simulink model "kay1024_recursive_demo"  (R2021b)
settings: Solver=FixedStepDiscrete  StartTime=0.0  StopTime=420  FixedStep=1  RelTol=1e-3
InitFcn:
  | kay_demo_init;
undefined symbols (not defined in the file or in its folder): i
libraries: hdlBasic x1189, dspsrcs4 x16, vmcUtilities x1
(part 1 of 14)
settings Model: Creator=Administrator  LastModifiedBy=Administrator

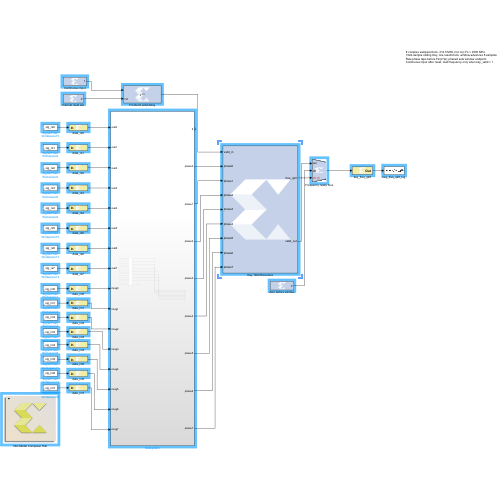
[thumbnail: Simulink's stored preview of the top-level diagram]
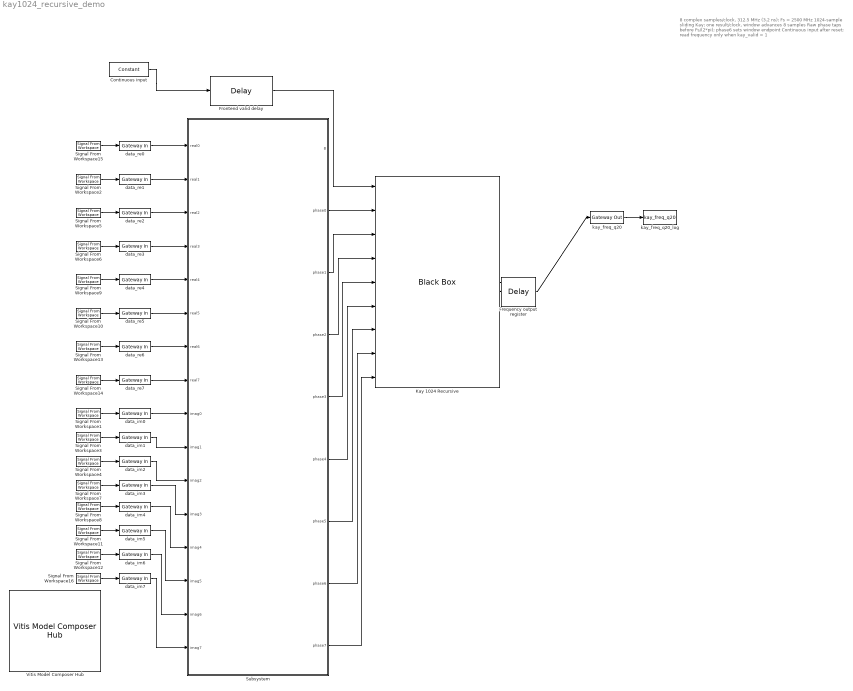
== system kay1024_recursive_demo ==
  note: 8 complex samples/clock, 312.5 MHz (3.2 ns); Fs = 2500 MHz
      | 1024-sample sliding Kay; one result/clock, window advances 8 samples
      | Raw phase taps before Fs/(2*pi); phase6 sets window endpoint
      | Continuous input after reset; read frequency only when kay_valid = 1
  Continuous input : hdlBasic/Constant  const=1  gui_display_data_type=Boolean  arith_type=Boolean  n_bits=16  bin_pt=14  preci_type=Single  exp_width=8  frac_width=24  explicit_period=on  period=1  XmcBlockStatus=1  maskContainerNames=tabcontainer1  block_type=constant  block_config=sysgen:Constant_config
  Frequency output register : hdlBasic/Delay  rst=off  en=off  latency=1  reg_retiming=off  XmcBlockStatus=1  maskContainerNames=group1  block_type=delay  block_config=sysgen:Delay_config
  Frontend valid delay : hdlBasic/Delay  rst=off  en=off  latency=23  reg_retiming=off  XmcBlockStatus=1  maskContainerNames=group1  block_type=delay  block_config=sysgen:Delay_config
  Kay 1024 Recursive : hdlBasic/Black Box  init_code=kay1024_phase_blackbox_config  sim_method=Vivado Simulator  verbose=off  XmcBlockStatus=1  maskContainerNames=group1  block_type=blackbox2  block_config=sysgen:black_box_config
  Signal From Workspace1 : dspsrcs4/Signal From Workspace  X=sig_im0  Ts=1  nsamps=1  OutputAfterFinalValue=Setting to zero  ignoreOrWarnInputAndFrameLengths=off  OutputFrames=on
  Signal From Workspace10 : dspsrcs4/Signal From Workspace  X=sig_re5  Ts=1  nsamps=1  OutputAfterFinalValue=Setting to zero  ignoreOrWarnInputAndFrameLengths=off  OutputFrames=on
  Signal From Workspace11 : dspsrcs4/Signal From Workspace  X=sig_im5  Ts=1  nsamps=1  OutputAfterFinalValue=Setting to zero  ignoreOrWarnInputAndFrameLengths=off  OutputFrames=on
  Signal From Workspace12 : dspsrcs4/Signal From Workspace  X=sig_im6  Ts=1  nsamps=1  OutputAfterFinalValue=Setting to zero  ignoreOrWarnInputAndFrameLengths=off  OutputFrames=on
  Signal From Workspace13 : dspsrcs4/Signal From Workspace  X=sig_re6  Ts=1  nsamps=1  OutputAfterFinalValue=Setting to zero  ignoreOrWarnInputAndFrameLengths=off  OutputFrames=on
  Signal From Workspace14 : dspsrcs4/Signal From Workspace  X=sig_re7  Ts=1  nsamps=1  OutputAfterFinalValue=Setting to zero  ignoreOrWarnInputAndFrameLengths=off  OutputFrames=on
  Signal From Workspace15 : dspsrcs4/Signal From Workspace  X=sig_re0  Ts=1  nsamps=1  OutputAfterFinalValue=Setting to zero  ignoreOrWarnInputAndFrameLengths=off  OutputFrames=on
  Signal From Workspace16 : dspsrcs4/Signal From Workspace  X=sig_im7  Ts=1  nsamps=1  OutputAfterFinalValue=Setting to zero  ignoreOrWarnInputAndFrameLengths=off  OutputFrames=on
  Signal From Workspace2 : dspsrcs4/Signal From Workspace  X=sig_re1  Ts=1  nsamps=1  OutputAfterFinalValue=Setting to zero  ignoreOrWarnInputAndFrameLengths=off  OutputFrames=on
  Signal From Workspace3 : dspsrcs4/Signal From Workspace  X=sig_im1  Ts=1  nsamps=1  OutputAfterFinalValue=Setting to zero  ignoreOrWarnInputAndFrameLengths=off  OutputFrames=on
  Signal From Workspace4 : dspsrcs4/Signal From Workspace  X=sig_im2  Ts=1  nsamps=1  OutputAfterFinalValue=Setting to zero  ignoreOrWarnInputAndFrameLengths=off  OutputFrames=on
  Signal From Workspace5 : dspsrcs4/Signal From Workspace  X=sig_re2  Ts=1  nsamps=1  OutputAfterFinalValue=Setting to zero  ignoreOrWarnInputAndFrameLengths=off  OutputFrames=on
  Signal From Workspace6 : dspsrcs4/Signal From Workspace  X=sig_re3  Ts=1  nsamps=1  OutputAfterFinalValue=Setting to zero  ignoreOrWarnInputAndFrameLengths=off  OutputFrames=on
  Signal From Workspace7 : dspsrcs4/Signal From Workspace  X=sig_im3  Ts=1  nsamps=1  OutputAfterFinalValue=Setting to zero  ignoreOrWarnInputAndFrameLengths=off  OutputFrames=on
  Signal From Workspace8 : dspsrcs4/Signal From Workspace  X=sig_im4  Ts=1  nsamps=1  OutputAfterFinalValue=Setting to zero  ignoreOrWarnInputAndFrameLengths=off  OutputFrames=on
  Signal From Workspace9 : dspsrcs4/Signal From Workspace  X=sig_re4  Ts=1  nsamps=1  OutputAfterFinalValue=Setting to zero  ignoreOrWarnInputAndFrameLengths=off  OutputFrames=on
  Subsystem : Subsystem
  Vitis Model Composer Hub : vmcUtilities/Vitis Model Composer Hub  Tag=genX  CodeGeneration=off  TargetDirectory=E:\FPGA\kay_recursive\build\sysgen  ExportType=System Generator  IpVendor=xilinx.com  IpLibrary=hls  IpVersion=1.0  IpHWLanguage=Verilog  AieCompilerOptions={}  CreateTestbench=off  TestbenchStackSize=10  RunAieSim=off  AieSimTimeout=50000  RunAieSimProfiling=off  LaunchVitisAnalyzer=off  PlotOutput=off  RunX86Sim=off  X86SimTimeout=10  GenHwImage=off  PlatformType=Not Specified  HwSystemType=Baremetal  HwValidationTarget=hw  ProjDevice=xczu47dr-ffve1156-2-i  ProjDevicePart=xczu47dr-ffve1156-2-i  SamplePeriod=-1  ClockFrequency=312.5  DataPathParallelism=1  xilinxfamily=zynquplusRFSOC  part=xczu47dr  speed=-2-i  package=ffve1156  directory=E:\FPGA\kay_recursive\build\sysgen  testbench=off  incr_netlist=off  synthesis_tool=Vivado  clock_wrapper=Clock Enables  dbl_ovrd=According to Block Masks  dcm_input_clock_period=10  sysclk_period=3.2  simulink_period=1  eval_field=0  IPInfoJsonString="{\"HDLSubsystem\":{\"SubsystemName\":\"kay1024_recursive_demo\",\"IPName\":\"kay1024_recursive\",\"IPLibrary\":\"user\",\"IPVendor\":\"user\",\"IPVersion\":\"1.0\"}}"
  data_im{0..7} (8 alike) : hdlBasic/Gateway In  gui_display_data_type=Fixed-point  arith_type=Signed (2's comp)  n_bits=14  bin_pt=13  preci_type=Single  exp_width=8  frac_width=24  rows=1  columns=1  quantization="Round  (unbiased: +/- Inf)"  overflow=Saturate  period=1  UseAsADC=off  ADCChannel='1'  interface=None  automatic_assignment=on  address_offset=hex2dec('00')  intf_name=''  intf_description=''  default_value=0  timing_constraint=None  locs_specified=off  LOCs={}  io_standard={}  inherit_from_input=off  hdl_port=on  XmcBlockStatus=1  maskContainerNames=group4  block_type=gatewayin  block_config=sysgen:gateway_in_config  block_width_w=590  block_height_w=620  block_width=640  block_height=850
  data_re{0..7} (8 alike) : hdlBasic/Gateway In  gui_display_data_type=Fixed-point  arith_type=Signed (2's comp)  n_bits=14  bin_pt=13  preci_type=Single  exp_width=8  frac_width=24  rows=1  columns=1  quantization="Round  (unbiased: +/- Inf)"  overflow=Saturate  period=1  UseAsADC=off  ADCChannel='1'  interface=None  automatic_assignment=on  address_offset=hex2dec('00')  intf_name=''  intf_description=''  default_value=0  timing_constraint=None  locs_specified=off  LOCs={}  io_standard={}  inherit_from_input=off  hdl_port=on  XmcBlockStatus=1  maskContainerNames=group4  block_type=gatewayin  block_config=sysgen:gateway_in_config  block_width_w=590  block_height_w=620  block_width=640  block_height=850
  kay_freq_q20 : hdlBasic/Gateway Out  inherit_from_input=off  hdl_port=on  rows=1  columns=1  UseAsDAC=off  DACChannel='1'  interface=None  automatic_assignment=on  address_offset=hex2dec('00')  intf_name=''  intf_description=''  timing_constraint=None  locs_specified=off  LOCs={}  io_standard={}  XmcBlockStatus=1  maskContainerNames=group4  block_type=gatewayout  block_config=sysgen:gateway_out_config  block_width_w=590  block_height_w=620  block_width=620  block_height=750
  kay_freq_q20_log : ToWorkspace  VariableName=kay_freq_q20  SaveFormat=Timeseries  SampleTime=-1
  wires:
  Subsystem/4(phase2) -> Kay 1024 Recursive/4
  Continuous input/1 -> Frontend valid delay/1
  Frequency output register/1 -> kay_freq_q20/1
  Signal From Workspace6/1 -> data_re3/1
  Subsystem/9(phase7) -> Kay 1024 Recursive/9
  Subsystem/5(phase3) -> Kay 1024 Recursive/5
  data_re1/1 -> Subsystem/2(real1)
  data_im5/1 -> Subsystem/14(imag5)
  Frontend valid delay/1 -> Kay 1024 Recursive/1
  Subsystem/7(phase5) -> Kay 1024 Recursive/7
  Subsystem/3(phase1) -> Kay 1024 Recursive/3
  Signal From Workspace9/1 -> data_re4/1
  Subsystem/8(phase6) -> Kay 1024 Recursive/8
  Signal From Workspace12/1 -> data_im6/1
  Signal From Workspace8/1 -> data_im4/1
  Subsystem/6(phase4) -> Kay 1024 Recursive/6
  Signal From Workspace2/1 -> data_re1/1
  Signal From Workspace13/1 -> data_re6/1
  Signal From Workspace1/1 -> data_im0/1
  Signal From Workspace5/1 -> data_re2/1
  kay_freq_q20/1 -> kay_freq_q20_log/1
  data_re0/1 -> Subsystem/1(real0)
  data_re3/1 -> Subsystem/4(real3)
  Signal From Workspace7/1 -> data_im3/1
  data_re5/1 -> Subsystem/6(real5)
  data_re6/1 -> Subsystem/7(real6)
  data_im2/1 -> Subsystem/11(imag2)
  data_im7/1 -> Subsystem/16(imag7)
  data_im6/1 -> Subsystem/15(imag6)
  Subsystem/2(phase0) -> Kay 1024 Recursive/2
  data_im3/1 -> Subsystem/12(imag3)
  Signal From Workspace10/1 -> data_re5/1
  Kay 1024 Recursive/1 -> Frequency output register/1
  data_im1/1 -> Subsystem/10(imag1)
  Signal From Workspace16/1 -> data_im7/1
  Signal From Workspace4/1 -> data_im2/1
  data_re4/1 -> Subsystem/5(real4)
  Signal From Workspace3/1 -> data_im1/1
  Signal From Workspace15/1 -> data_re0/1
  Signal From Workspace14/1 -> data_re7/1
  data_re7/1 -> Subsystem/8(real7)
  Signal From Workspace11/1 -> data_im5/1
  data_im0/1 -> Subsystem/9(imag0)
  data_re2/1 -> Subsystem/3(real2)
  data_im4/1 -> Subsystem/13(imag4)

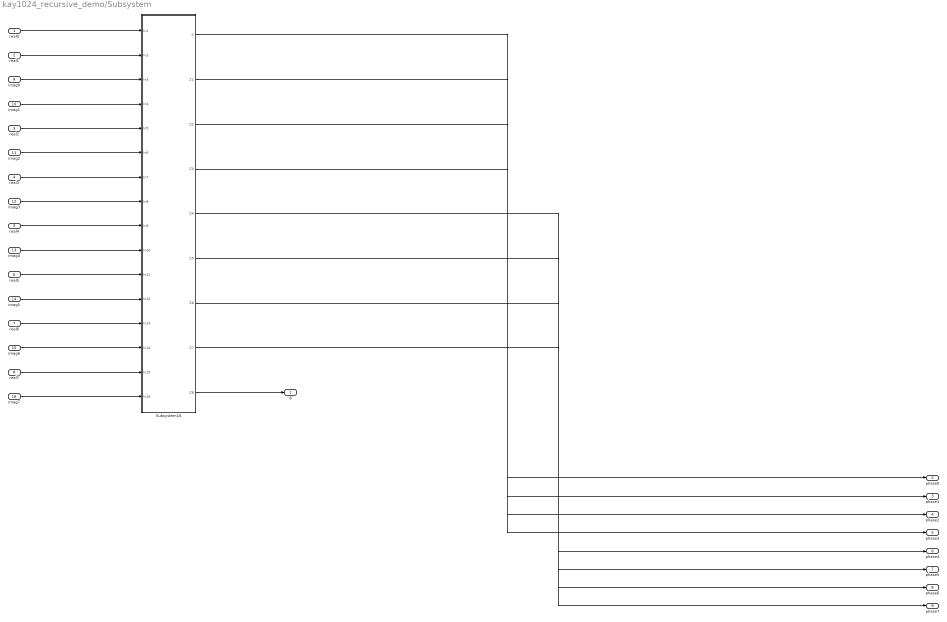
== system kay1024_recursive_demo/Subsystem ==
  real0 : Inport
  real1 : Inport  Port=2
  real2 : Inport  Port=3
  real3 : Inport  Port=4
  real4 : Inport  Port=5
  real5 : Inport  Port=6
  real6 : Inport  Port=7
  real7 : Inport  Port=8
  imag0 : Inport  Port=9
  imag1 : Inport  Port=10
  imag2 : Inport  Port=11
  imag3 : Inport  Port=12
  imag4 : Inport  Port=13
  imag5 : Inport  Port=14
  imag6 : Inport  Port=15
  imag7 : Inport  Port=16
  Subsystem16 : Subsystem
  8 : Outport
  phase0 : Outport  Port=2
  phase1 : Outport  Port=3
  phase2 : Outport  Port=4
  phase3 : Outport  Port=5
  phase4 : Outport  Port=6
  phase5 : Outport  Port=7
  phase6 : Outport  Port=8
  phase7 : Outport  Port=9
  wires:
  real0/1 -> Subsystem16/1(In1)
  real1/1 -> Subsystem16/2(In2)
  imag0/1 -> Subsystem16/3(In3)
  imag1/1 -> Subsystem16/4(In4)
  real2/1 -> Subsystem16/5(In5)
  imag2/1 -> Subsystem16/6(In6)
  real3/1 -> Subsystem16/7(In7)
  imag3/1 -> Subsystem16/8(In8)
  real4/1 -> Subsystem16/9(In9)
  imag4/1 -> Subsystem16/10(In10)
  real5/1 -> Subsystem16/11(In11)
  imag5/1 -> Subsystem16/12(In12)
  real6/1 -> Subsystem16/13(In13)
  imag6/1 -> Subsystem16/14(In14)
  real7/1 -> Subsystem16/15(In15)
  imag7/1 -> Subsystem16/16(In16)
  Subsystem16/8(Z7) -> phase7/1
  Subsystem16/7(Z6) -> phase6/1
  Subsystem16/6(Z5) -> phase5/1
  Subsystem16/5(Z4) -> phase4/1
  Subsystem16/3(Z2) -> phase2/1
  Subsystem16/2(Z1) -> phase1/1
  Subsystem16/4(Z3) -> phase3/1
  Subsystem16/1(Z) -> phase0/1
  Subsystem16/9(Z8) -> 8/1

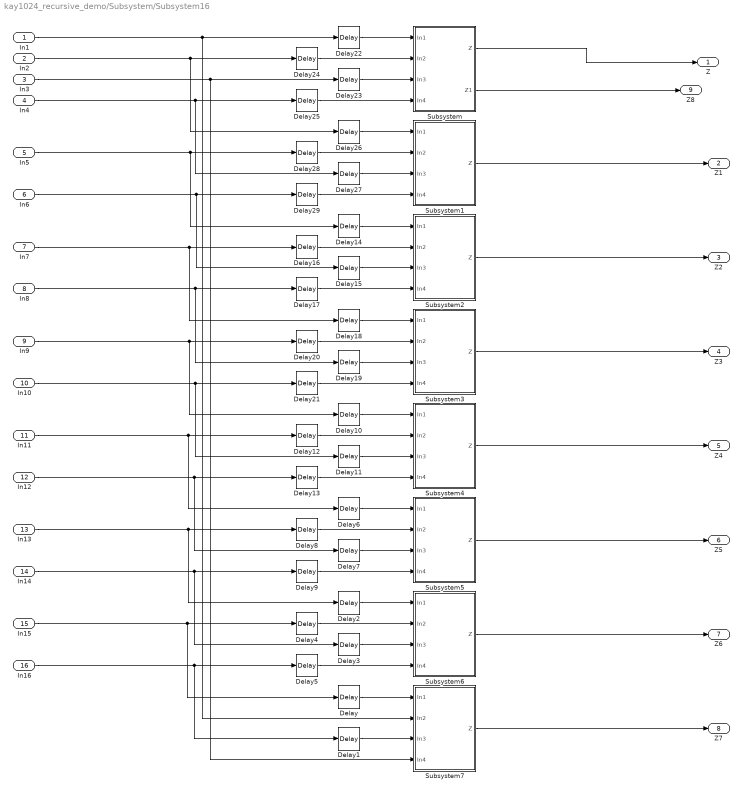
== system kay1024_recursive_demo/Subsystem/Subsystem16 ==
  In1 : Inport
  In2 : Inport  Port=2
  In3 : Inport  Port=3
  In4 : Inport  Port=4
  In5 : Inport  Port=5
  In6 : Inport  Port=6
  In7 : Inport  Port=7
  In8 : Inport  Port=8
  In9 : Inport  Port=9
  In10 : Inport  Port=10
  In11 : Inport  Port=11
  In12 : Inport  Port=12
  In13 : Inport  Port=13
  In14 : Inport  Port=14
  In15 : Inport  Port=15
  In16 : Inport  Port=16
  Delay{,1..29} (30 alike) : hdlBasic/Delay  rst=off  en=off  latency=1  reg_retiming=off  XmcBlockStatus=1  maskContainerNames=group1  block_type=delay  block_config=sysgen:Delay_config
  Subsystem : Subsystem
  Subsystem1 : Subsystem
  Subsystem2 : Subsystem
  Subsystem3 : Subsystem
  Subsystem4 : Subsystem
  Subsystem5 : Subsystem
  Subsystem6 : Subsystem
  Subsystem7 : Subsystem
  Z : Outport
  Z1 : Outport  Port=2
  Z2 : Outport  Port=3
  Z3 : Outport  Port=4
  Z4 : Outport  Port=5
  Z5 : Outport  Port=6
  Z6 : Outport  Port=7
  Z7 : Outport  Port=8
  Z8 : Outport  Port=9
  wires:
  In3/1 -> Subsystem7/4(In4), Delay23/1
  In16/1 -> Delay5/1, Delay1/1
  In1/1 -> Subsystem7/2(In2), Delay22/1
  In11/1 -> Delay12/1, Delay6/1
  In6/1 -> Delay15/1, Delay29/1
  In4/1 -> Delay27/1, Delay25/1
  In13/1 -> Delay2/1, Delay8/1
  In9/1 -> Delay10/1, Delay20/1
  In7/1 -> Delay18/1, Delay16/1
  In8/1 -> Delay19/1, Delay17/1
  In12/1 -> Delay7/1, Delay13/1
  In2/1 -> Delay26/1, Delay24/1
  Subsystem5/1(Z) -> Z5/1
  Subsystem7/1(Z) -> Z7/1
  In5/1 -> Delay14/1, Delay28/1
  Subsystem1/1(Z) -> Z1/1
  In14/1 -> Delay3/1, Delay9/1
  In10/1 -> Delay11/1, Delay21/1
  In15/1 -> Delay4/1, Delay/1
  Subsystem/1(Z) -> Z/1
  Subsystem4/1(Z) -> Z4/1
  Subsystem6/1(Z) -> Z6/1
  Subsystem2/1(Z) -> Z2/1
  Subsystem3/1(Z) -> Z3/1
  Delay/1 -> Subsystem7/1(In1)
  Delay1/1 -> Subsystem7/3(In3)
  Delay3/1 -> Subsystem6/3(In3)
  Delay2/1 -> Subsystem6/1(In1)
  Delay4/1 -> Subsystem6/2(In2)
  Delay5/1 -> Subsystem6/4(In4)
  Delay9/1 -> Subsystem5/4(In4)
  Delay7/1 -> Subsystem5/3(In3)
  Delay8/1 -> Subsystem5/2(In2)
  Delay6/1 -> Subsystem5/1(In1)
  Delay13/1 -> Subsystem4/4(In4)
  Delay10/1 -> Subsystem4/1(In1)
  Delay12/1 -> Subsystem4/2(In2)
  Delay11/1 -> Subsystem4/3(In3)
  Delay15/1 -> Subsystem2/3(In3)
  Delay16/1 -> Subsystem2/2(In2)
  Delay14/1 -> Subsystem2/1(In1)
  Delay21/1 -> Subsystem3/4(In4)
  Delay19/1 -> Subsystem3/3(In3)
  Delay20/1 -> Subsystem3/2(In2)
  Delay17/1 -> Subsystem2/4(In4)
  Delay18/1 -> Subsystem3/1(In1)
  Delay26/1 -> Subsystem1/1(In1)
  Delay27/1 -> Subsystem1/3(In3)
  Delay28/1 -> Subsystem1/2(In2)
  Delay29/1 -> Subsystem1/4(In4)
  Delay23/1 -> Subsystem/3(In3)
  Delay24/1 -> Subsystem/2(In2)
  Delay22/1 -> Subsystem/1(In1)
  Delay25/1 -> Subsystem/4(In4)
  Subsystem/2(Z1) -> Z8/1

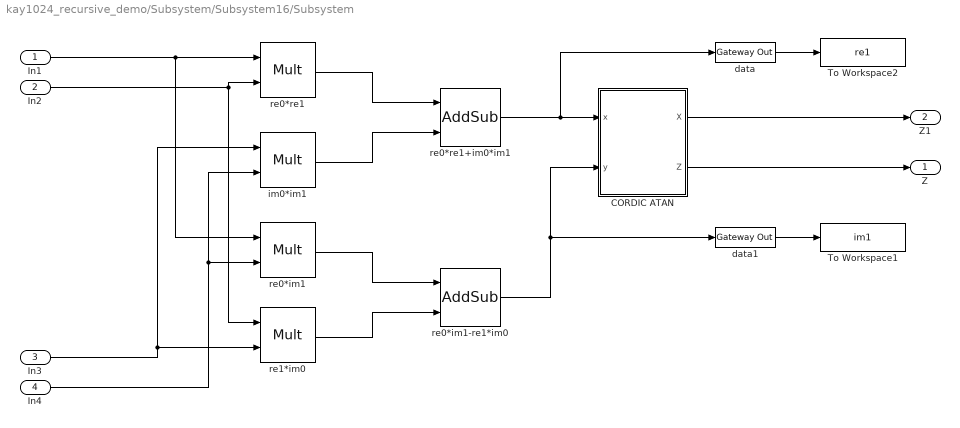
== system kay1024_recursive_demo/Subsystem/Subsystem16/Subsystem ==
  In1 : Inport
  In2 : Inport  Port=2
  In3 : Inport  Port=3
  In4 : Inport  Port=4
  CORDIC ATAN : Subsystem  mask(Xilinx CORDIC ATAN){stages=15, pe_nbits=30, pe_binpt=18, pipeline_x=ones(1,15), prev_stages=15, pipeline=[1  1  1  1  1  1  1  1  1  1  1  1  1  1  1]}
      mask prompts: stages "Number of Processing Elements (integer value starting from 1)"; pe_nbits "X, Y Data Width"; pe_binpt "X, Y Binary Point Position"; pipeline_x "Latency for each Processing Element [1 0 0 1]"; prev_stages "Previous Number of Stages"; pipeline "Previous Pipeline Values"
      mask help: A parallel implementation, circular vectoring mode CORDIC processor for performing rectangular-to-polar conversion. The number of iteration stages (and resultant output accuracy) and the processor arithmetic precision are controlled by the mask customization.
      mask init:
      | [bg,fg] = xlcmap('XBlock',0);
      | iPos = get_param(gcb,'Position');
      | iWidth=iPos(3)-iPos(1); iHeight=iPos(4)-iPos(2);
      | iCx=iWidth/2;
      | iCy=iHeight/2;
      | [logoX, logoY] = xlogo(iPos);
      | sav_gcb=gcb;
      | stages = round(sum(abs(stages)));
      | if (stages == 0)
      | 	stages = prev_stages;
      | end
      | x = zeros(1,stages);
      | pipe_size = max(size(pipeline_x));
      | if pipe_size >= stages
      | 	x(1,1:stages) = pipeline_x(1,1:stages);
      | else
      | 	x(1,1:pipe_size) = pipeline_x(1,1:pipe_size);
      | end
      | 
      | if (stages ~=prev_stages)
      | 	pipeline=x;
      | 	cordic_pe = find_system(gcb, 'lookUnderMasks', 'all', 'FollowLinks','on','masktype', 'CORDIC parallel PE');
      |     
      |   a=find_system(cordic_pe{1}, 'lookUnderMasks', 'all', 'FollowLinks','on','masktype', 'CORDIC iteration PE');
      |   for i= 2:length(a)
      |     for j=1:3
      | 	  delete_line(cordic_pe{1}, ['CORDIC PE' int2str(i-1) '/' int2str(j)], ['CORDIC PE' int2str(i) '/' int2str(j)]);
      |     end
      |   end
      |     if length(a)>0,
      |       delete_line(cordic_pe{1}, 'x/1', 'CORDIC PE1/1');
      |       delete_line(cordic_pe{1}, 'y/1', 'CORDIC PE1/2');
      |       delete_line(cordic_pe{1}, 'z/1', 'CORDIC PE1/3');
      |       delete_line(cordic_pe{1}, ['CORDIC PE' int2str(length(a)) '/1'],'X/1');
      |       delete_line(cordic_pe{1}, ['CORDIC PE' int2str(length(a)) '/2'],'Terminator/1');
      |       delete_line(cordic_pe{1}, ['CORDIC PE' int2str(length(a)) '/3'],'Z/1');
      |     elseif length(a)==0
      |       temp_port=get_param([cordic_pe{1} '/x'],'porthandles');
      |       temp_line=get_param(temp_port.Outport,'line');
      |       if temp_line>=0  delete_line(temp_line); end
      |       temp_port=get_param([cordic_pe{1} '/y'],'porthandles');
      |       temp_line=get_param(temp_port.Outport,'line');
      |       if temp_line>=0  delete_line(temp_line); end
      |       temp_port=get_param([cordic_pe{1} '/z'],'porthandles');
      |       temp_line=get_param(temp_port.Outport,'line');
      |       if temp_line>=0  delete_line(temp_line); end
      |     end
      | 
      |     for i=2:length(a)
      |       delete_block(a{i});
      |     end
      |     for i=2:stages,
      |         add_block([cordic_pe{1} '/CORDIC PE1'], [cordic_pe{1} '/CORDIC PE' int2str(i)], 'ii', int2str(i-1),'pe_nbits', 'pe_nbits','pe_binpt', 'pe_binpt','pipeline',['pipeline(1,' int2str(i) ')'],'position',[150+(i-1)*125, 70, 205+(i-1)*125, 130]);
      |     end
      | 
      |     for i= 2:stages,
      |       for j=1:3
      | 		add_line(cordic_pe{1}, ['CORDIC PE' int2str(i-1) '/' int2str(j)], ['CORDIC PE' int2str(i) '/' int2str(j)], 'autorouting', 'on');
      |       end
      |     end
      | 
      |     if stages==0
      |       add_line(cordic_pe{1}, 'x/1', 'X/1', 'autorouting', 'on');
      |       add_line(cordic_pe{1}, 'y/1', 'Terminator/1', 'autorouting', 'on');
      |       add_line(cordic_pe{1}, 'z/1', 'Z/1', 'autorouting', 'on');
      |     elseif stages>0
      |       add_line(cordic_pe{1}, 'x/1', 'CORDIC PE1/1', 'autorouting', 'on');
      |       add_line(cordic_pe{1}, 'y/1', 'CORDIC PE1/2', 'autorouting', 'on');
      |       add_line(cordic_pe{1}, 'z/1', 'CORDIC PE1/3', 'autorouting', 'on');
      | 
      |       set_param([cordic_pe{1} '/' 'X'], 'Position', [150+stages*125, 72, 180+stages*125, 86]);
      |       set_param([cordic_pe{1} '/' 'Terminator'], 'Position', [210+stages*125, 92, 225+stages*125, 108]);
      |       set_param([cordic_pe{1} '/' 'Z'], 'Position', [240+stages*125, 113, 270+stages*125, 127]);
      | 
      |       add_line(cordic_pe{1}, ['CORDIC PE' int2str(stages) '/1'], 'X/1', 'autorouting', 'on');
      |       add_line(cordic_pe{1}, ['CORDIC PE' int2str(stages) '/2'], 'Terminator/1', 'autorouting', 'on');
      |       add_line(cordic_pe{1}, ['CORDIC PE' int2str(stages) '/3'],'Z/1', 'autorouting', 'on');
      | 
      |       % force a "compile" of the constituent constant blocks to
      |       % workaround a data propagation problem
      |       find_system(cordic_pe{1}, 'lookUnderMasks', 'all', 'FollowLinks', 'on', 'MaskType','Xilinx Constant Block');
      |   end
      | 	set_param(sav_gcb, 'prev_stages', int2str(stages));
      | 	set_param(sav_gcb, 'pipeline', [ '[' int2str(x) ']']);
      | else
      | 	if (sum(pipeline~=x))
      | 		set_param(gcb, 'pipeline', [ '[' int2str(x) ']']);
      | 	end
      | end
      | str = sprintf('-%d',sum(x) + 3);
      settings: CopyFcn=set_param(gcb, 'MaskSelfModifiable', 'on', 'LinkStatus', 'none');
      mask Help: eval('');xlDoc('-book','sysgen','-topic','CORDIC_ATAN');
      mask Display:
      | patch([0 iWidth iWidth 0],[0 0 iHeight iHeight] , bg);
      | patch(logoX,logoY , fg);
      | text(iCx-6,iCy,'z');
      | text(iCx,iCy+4,str);
      | port_label('input',1,'x');
      | port_label('input',2,'y');
      | port_label('output',1,'mag');
      | port_label('output',2,'atan');
      | plot([0 0 iWidth iWidth 0], [0 iHeight iHeight 0 0]);
  To Workspace1 : ToWorkspace  VariableName=im1  SampleTime=-1
      settings: Save2DSignal=2-D array (concatenate along first dimension)
  To Workspace2 : ToWorkspace  VariableName=re1  SampleTime=-1
      settings: Save2DSignal=2-D array (concatenate along first dimension)
  data : hdlBasic/Gateway Out  inherit_from_input=on  hdl_port=off  rows=1  columns=1  UseAsDAC=off  DACChannel='1'  interface=None  automatic_assignment=on  address_offset=hex2dec('00')  intf_name=''  intf_description=''  timing_constraint=None  locs_specified=off  LOCs={}  io_standard={}  XmcBlockStatus=1  maskContainerNames=group4  block_type=gatewayout  block_config=sysgen:gateway_out_config  block_width_w=590  block_height_w=620  block_width=620  block_height=750
  data1 : hdlBasic/Gateway Out  inherit_from_input=on  hdl_port=off  rows=1  columns=1  UseAsDAC=off  DACChannel='1'  interface=None  automatic_assignment=on  address_offset=hex2dec('00')  intf_name=''  intf_description=''  timing_constraint=None  locs_specified=off  LOCs={}  io_standard={}  XmcBlockStatus=1  maskContainerNames=group4  block_type=gatewayout  block_config=sysgen:gateway_out_config  block_width_w=590  block_height_w=620  block_width=620  block_height=750
  im0*im1 : hdlBasic/Mult  precision=Full  arith_type="Signed  (2's comp)"  n_bits=16  bin_pt=14  quantization=Truncate  overflow=Wrap  en=off  latency=3  use_behavioral_HDL=off  opt=Speed  use_embedded=on  optimum_pipeline=off  pipeline=on  use_rpm=on  placement_style=Triangular  XmcBlockStatus=1  maskContainerNames=group1  block_type=mult  block_config=sysgen:Mult_config  block_width=598  block_height=876
  re0*im1 : hdlBasic/Mult  precision=Full  arith_type="Signed  (2's comp)"  n_bits=16  bin_pt=14  quantization=Truncate  overflow=Wrap  en=off  latency=3  use_behavioral_HDL=off  opt=Speed  use_embedded=on  optimum_pipeline=off  pipeline=on  use_rpm=on  placement_style=Triangular  XmcBlockStatus=1  maskContainerNames=group1  block_type=mult  block_config=sysgen:Mult_config  block_width=598  block_height=876
  re0*im1-re1*im0 : hdlBasic/AddSub  mode=Subtraction  use_carryin=off  use_carryout=off  en=off  latency=1  precision=Full  arith_type=Unsigned  n_bits=16  bin_pt=14  quantization=Truncate  overflow=Wrap  use_behavioral_HDL=off  hw_selection=Fabric  pipelined=off  XmcBlockStatus=1  maskContainerNames=tabcontainer1  block_type=addsub  block_config=sysgen:Addsub_config
  re0*re1 : hdlBasic/Mult  precision=Full  arith_type="Signed  (2's comp)"  n_bits=16  bin_pt=14  quantization=Truncate  overflow=Wrap  en=off  latency=3  use_behavioral_HDL=off  opt=Speed  use_embedded=on  optimum_pipeline=off  pipeline=on  use_rpm=on  placement_style=Triangular  XmcBlockStatus=1  maskContainerNames=group1  block_type=mult  block_config=sysgen:Mult_config  block_width=598  block_height=876
  re0*re1+im0*im1 : hdlBasic/AddSub  mode=Addition  use_carryin=off  use_carryout=off  en=off  latency=1  precision=Full  arith_type=Unsigned  n_bits=16  bin_pt=14  quantization=Truncate  overflow=Wrap  use_behavioral_HDL=off  hw_selection=Fabric  pipelined=off  XmcBlockStatus=1  maskContainerNames=tabcontainer1  block_type=addsub  block_config=sysgen:Addsub_config
  re1*im0 : hdlBasic/Mult  precision=Full  arith_type="Signed  (2's comp)"  n_bits=16  bin_pt=14  quantization=Truncate  overflow=Wrap  en=off  latency=3  use_behavioral_HDL=off  opt=Speed  use_embedded=on  optimum_pipeline=off  pipeline=on  use_rpm=on  placement_style=Triangular  XmcBlockStatus=1  maskContainerNames=group1  block_type=mult  block_config=sysgen:Mult_config  block_width=598  block_height=876
  Z : Outport
  Z1 : Outport  Port=2
  wires:
  In3/1 -> re1*im0/2, im0*im1/1
  re0*im1-re1*im0/1 -> CORDIC ATAN/2(y), data1/1
  In2/1 -> re0*re1/2, re1*im0/1
  In4/1 -> re0*im1/2, im0*im1/2
  re0*im1/1 -> re0*im1-re1*im0/1
  In1/1 -> re0*im1/1, re0*re1/1
  re0*re1/1 -> re0*re1+im0*im1/1
  im0*im1/1 -> re0*re1+im0*im1/2
  re0*re1+im0*im1/1 -> data/1, CORDIC ATAN/1(x)
  re1*im0/1 -> re0*im1-re1*im0/2
  CORDIC ATAN/2(Z) -> Z/1
  data/1 -> To Workspace2/1
  data1/1 -> To Workspace1/1
  CORDIC ATAN/1(X) -> Z1/1

== system kay1024_recursive_demo/Subsystem/Subsystem16/Subsystem1 ==
  In1 : Inport
  In2 : Inport  Port=2
  In3 : Inport  Port=3
  In4 : Inport  Port=4
  CORDIC ATAN : Subsystem  mask(Xilinx CORDIC ATAN){stages=15, pe_nbits=30, pe_binpt=18, pipeline_x=ones(1,15), prev_stages=15, pipeline=[1  1  1  1  1  1  1  1  1  1  1  1  1  1  1]}
      mask prompts: stages "Number of Processing Elements (integer value starting from 1)"; pe_nbits "X, Y Data Width"; pe_binpt "X, Y Binary Point Position"; pipeline_x "Latency for each Processing Element [1 0 0 1]"; prev_stages "Previous Number of Stages"; pipeline "Previous Pipeline Values"
      mask help: A parallel implementation, circular vectoring mode CORDIC processor for performing rectangular-to-polar conversion. The number of iteration stages (and resultant output accuracy) and the processor arithmetic precision are controlled by the mask customization.
      mask init: same as kay1024_recursive_demo/Subsystem/Subsystem16/Subsystem/CORDIC ATAN
      settings: CopyFcn=set_param(gcb, 'MaskSelfModifiable', 'on', 'LinkStatus', 'none');
      mask Help: eval('');xlDoc('-book','sysgen','-topic','CORDIC_ATAN');
      mask Display:
      | patch([0 iWidth iWidth 0],[0 0 iHeight iHeight] , bg);
      | patch(logoX,logoY , fg);
      | text(iCx-6,iCy,'z');
      | text(iCx,iCy+4,str);
      | port_label('input',1,'x');
      | port_label('input',2,'y');
      | port_label('output',1,'mag');
      | port_label('output',2,'atan');
      | plot([0 0 iWidth iWidth 0], [0 iHeight iHeight 0 0]);
  im0*im1 : hdlBasic/Mult  precision=Full  arith_type="Signed  (2's comp)"  n_bits=16  bin_pt=14  quantization=Truncate  overflow=Wrap  en=off  latency=3  use_behavioral_HDL=off  opt=Speed  use_embedded=on  optimum_pipeline=off  pipeline=on  use_rpm=on  placement_style=Triangular  XmcBlockStatus=1  maskContainerNames=group1  block_type=mult  block_config=sysgen:Mult_config  block_width=598  block_height=876
  re0*im1 : hdlBasic/Mult  precision=Full  arith_type="Signed  (2's comp)"  n_bits=16  bin_pt=14  quantization=Truncate  overflow=Wrap  en=off  latency=3  use_behavioral_HDL=off  opt=Speed  use_embedded=on  optimum_pipeline=off  pipeline=on  use_rpm=on  placement_style=Triangular  XmcBlockStatus=1  maskContainerNames=group1  block_type=mult  block_config=sysgen:Mult_config  block_width=598  block_height=876
  re0*im1-re1*im0 : hdlBasic/AddSub  mode=Subtraction  use_carryin=off  use_carryout=off  en=off  latency=1  precision=Full  arith_type=Unsigned  n_bits=16  bin_pt=14  quantization=Truncate  overflow=Wrap  use_behavioral_HDL=off  hw_selection=Fabric  pipelined=off  XmcBlockStatus=1  maskContainerNames=tabcontainer1  block_type=addsub  block_config=sysgen:Addsub_config
  re0*re1 : hdlBasic/Mult  precision=Full  arith_type="Signed  (2's comp)"  n_bits=16  bin_pt=14  quantization=Truncate  overflow=Wrap  en=off  latency=3  use_behavioral_HDL=off  opt=Speed  use_embedded=on  optimum_pipeline=off  pipeline=on  use_rpm=on  placement_style=Triangular  XmcBlockStatus=1  maskContainerNames=group1  block_type=mult  block_config=sysgen:Mult_config  block_width=598  block_height=876
  re0*re1+im0*im1 : hdlBasic/AddSub  mode=Addition  use_carryin=off  use_carryout=off  en=off  latency=1  precision=Full  arith_type=Unsigned  n_bits=16  bin_pt=14  quantization=Truncate  overflow=Wrap  use_behavioral_HDL=off  hw_selection=Fabric  pipelined=off  XmcBlockStatus=1  maskContainerNames=tabcontainer1  block_type=addsub  block_config=sysgen:Addsub_config
  re1*im0 : hdlBasic/Mult  precision=Full  arith_type="Signed  (2's comp)"  n_bits=16  bin_pt=14  quantization=Truncate  overflow=Wrap  en=off  latency=3  use_behavioral_HDL=off  opt=Speed  use_embedded=on  optimum_pipeline=off  pipeline=on  use_rpm=on  placement_style=Triangular  XmcBlockStatus=1  maskContainerNames=group1  block_type=mult  block_config=sysgen:Mult_config  block_width=598  block_height=876
  Z : Outport
  wires:
  In3/1 -> re1*im0/2, im0*im1/1
  re0*im1-re1*im0/1 -> CORDIC ATAN/2(y)
  In2/1 -> re0*re1/2, re1*im0/1
  In4/1 -> re0*im1/2, im0*im1/2
  re0*im1/1 -> re0*im1-re1*im0/1
  In1/1 -> re0*im1/1, re0*re1/1
  re0*re1/1 -> re0*re1+im0*im1/1
  im0*im1/1 -> re0*re1+im0*im1/2
  re0*re1+im0*im1/1 -> CORDIC ATAN/1(x)
  re1*im0/1 -> re0*im1-re1*im0/2
  CORDIC ATAN/2(Z) -> Z/1

== system kay1024_recursive_demo/Subsystem/Subsystem16/Subsystem2 ==
  In1 : Inport
  In2 : Inport  Port=2
  In3 : Inport  Port=3
  In4 : Inport  Port=4
  CORDIC ATAN : Subsystem  mask(Xilinx CORDIC ATAN){stages=15, pe_nbits=30, pe_binpt=18, pipeline_x=ones(1,15), prev_stages=15, pipeline=[1  1  1  1  1  1  1  1  1  1  1  1  1  1  1]}
      mask prompts: stages "Number of Processing Elements (integer value starting from 1)"; pe_nbits "X, Y Data Width"; pe_binpt "X, Y Binary Point Position"; pipeline_x "Latency for each Processing Element [1 0 0 1]"; prev_stages "Previous Number of Stages"; pipeline "Previous Pipeline Values"
      mask help: A parallel implementation, circular vectoring mode CORDIC processor for performing rectangular-to-polar conversion. The number of iteration stages (and resultant output accuracy) and the processor arithmetic precision are controlled by the mask customization.
      mask init: same as kay1024_recursive_demo/Subsystem/Subsystem16/Subsystem/CORDIC ATAN
      settings: CopyFcn=set_param(gcb, 'MaskSelfModifiable', 'on', 'LinkStatus', 'none');
      mask Help: eval('');xlDoc('-book','sysgen','-topic','CORDIC_ATAN');
      mask Display:
      | patch([0 iWidth iWidth 0],[0 0 iHeight iHeight] , bg);
      | patch(logoX,logoY , fg);
      | text(iCx-6,iCy,'z');
      | text(iCx,iCy+4,str);
      | port_label('input',1,'x');
      | port_label('input',2,'y');
      | port_label('output',1,'mag');
      | port_label('output',2,'atan');
      | plot([0 0 iWidth iWidth 0], [0 iHeight iHeight 0 0]);
  im0*im1 : hdlBasic/Mult  precision=Full  arith_type="Signed  (2's comp)"  n_bits=16  bin_pt=14  quantization=Truncate  overflow=Wrap  en=off  latency=3  use_behavioral_HDL=off  opt=Speed  use_embedded=on  optimum_pipeline=off  pipeline=on  use_rpm=on  placement_style=Triangular  XmcBlockStatus=1  maskContainerNames=group1  block_type=mult  block_config=sysgen:Mult_config  block_width=598  block_height=876
  re0*im1 : hdlBasic/Mult  precision=Full  arith_type="Signed  (2's comp)"  n_bits=16  bin_pt=14  quantization=Truncate  overflow=Wrap  en=off  latency=3  use_behavioral_HDL=off  opt=Speed  use_embedded=on  optimum_pipeline=off  pipeline=on  use_rpm=on  placement_style=Triangular  XmcBlockStatus=1  maskContainerNames=group1  block_type=mult  block_config=sysgen:Mult_config  block_width=598  block_height=876
  re0*im1-re1*im0 : hdlBasic/AddSub  mode=Subtraction  use_carryin=off  use_carryout=off  en=off  latency=1  precision=Full  arith_type=Unsigned  n_bits=16  bin_pt=14  quantization=Truncate  overflow=Wrap  use_behavioral_HDL=off  hw_selection=Fabric  pipelined=off  XmcBlockStatus=1  maskContainerNames=tabcontainer1  block_type=addsub  block_config=sysgen:Addsub_config
  re0*re1 : hdlBasic/Mult  precision=Full  arith_type="Signed  (2's comp)"  n_bits=16  bin_pt=14  quantization=Truncate  overflow=Wrap  en=off  latency=3  use_behavioral_HDL=off  opt=Speed  use_embedded=on  optimum_pipeline=off  pipeline=on  use_rpm=on  placement_style=Triangular  XmcBlockStatus=1  maskContainerNames=group1  block_type=mult  block_config=sysgen:Mult_config  block_width=598  block_height=876
  re0*re1+im0*im1 : hdlBasic/AddSub  mode=Addition  use_carryin=off  use_carryout=off  en=off  latency=1  precision=Full  arith_type=Unsigned  n_bits=16  bin_pt=14  quantization=Truncate  overflow=Wrap  use_behavioral_HDL=off  hw_selection=Fabric  pipelined=off  XmcBlockStatus=1  maskContainerNames=tabcontainer1  block_type=addsub  block_config=sysgen:Addsub_config
  re1*im0 : hdlBasic/Mult  precision=Full  arith_type="Signed  (2's comp)"  n_bits=16  bin_pt=14  quantization=Truncate  overflow=Wrap  en=off  latency=3  use_behavioral_HDL=off  opt=Speed  use_embedded=on  optimum_pipeline=off  pipeline=on  use_rpm=on  placement_style=Triangular  XmcBlockStatus=1  maskContainerNames=group1  block_type=mult  block_config=sysgen:Mult_config  block_width=598  block_height=876
  Z : Outport
  wires:
  In3/1 -> re1*im0/2, im0*im1/1
  re0*im1-re1*im0/1 -> CORDIC ATAN/2(y)
  In2/1 -> re0*re1/2, re1*im0/1
  In4/1 -> re0*im1/2, im0*im1/2
  re0*im1/1 -> re0*im1-re1*im0/1
  In1/1 -> re0*im1/1, re0*re1/1
  re0*re1/1 -> re0*re1+im0*im1/1
  im0*im1/1 -> re0*re1+im0*im1/2
  re0*re1+im0*im1/1 -> CORDIC ATAN/1(x)
  re1*im0/1 -> re0*im1-re1*im0/2
  CORDIC ATAN/2(Z) -> Z/1

== system kay1024_recursive_demo/Subsystem/Subsystem16/Subsystem3 ==
  In1 : Inport
  In2 : Inport  Port=2
  In3 : Inport  Port=3
  In4 : Inport  Port=4
  CORDIC ATAN : Subsystem  mask(Xilinx CORDIC ATAN){stages=15, pe_nbits=30, pe_binpt=18, pipeline_x=ones(1,15), prev_stages=15, pipeline=[1  1  1  1  1  1  1  1  1  1  1  1  1  1  1]}
      mask prompts: stages "Number of Processing Elements (integer value starting from 1)"; pe_nbits "X, Y Data Width"; pe_binpt "X, Y Binary Point Position"; pipeline_x "Latency for each Processing Element [1 0 0 1]"; prev_stages "Previous Number of Stages"; pipeline "Previous Pipeline Values"
      mask help: A parallel implementation, circular vectoring mode CORDIC processor for performing rectangular-to-polar conversion. The number of iteration stages (and resultant output accuracy) and the processor arithmetic precision are controlled by the mask customization.
      mask init: same as kay1024_recursive_demo/Subsystem/Subsystem16/Subsystem/CORDIC ATAN
      settings: CopyFcn=set_param(gcb, 'MaskSelfModifiable', 'on', 'LinkStatus', 'none');
      mask Help: eval('');xlDoc('-book','sysgen','-topic','CORDIC_ATAN');
      mask Display:
      | patch([0 iWidth iWidth 0],[0 0 iHeight iHeight] , bg);
      | patch(logoX,logoY , fg);
      | text(iCx-6,iCy,'z');
      | text(iCx,iCy+4,str);
      | port_label('input',1,'x');
      | port_label('input',2,'y');
      | port_label('output',1,'mag');
      | port_label('output',2,'atan');
      | plot([0 0 iWidth iWidth 0], [0 iHeight iHeight 0 0]);
  im0*im1 : hdlBasic/Mult  precision=Full  arith_type="Signed  (2's comp)"  n_bits=16  bin_pt=14  quantization=Truncate  overflow=Wrap  en=off  latency=3  use_behavioral_HDL=off  opt=Speed  use_embedded=on  optimum_pipeline=off  pipeline=on  use_rpm=on  placement_style=Triangular  XmcBlockStatus=1  maskContainerNames=group1  block_type=mult  block_config=sysgen:Mult_config  block_width=598  block_height=876
  re0*im1 : hdlBasic/Mult  precision=Full  arith_type="Signed  (2's comp)"  n_bits=16  bin_pt=14  quantization=Truncate  overflow=Wrap  en=off  latency=3  use_behavioral_HDL=off  opt=Speed  use_embedded=on  optimum_pipeline=off  pipeline=on  use_rpm=on  placement_style=Triangular  XmcBlockStatus=1  maskContainerNames=group1  block_type=mult  block_config=sysgen:Mult_config  block_width=598  block_height=876
  re0*im1-re1*im0 : hdlBasic/AddSub  mode=Subtraction  use_carryin=off  use_carryout=off  en=off  latency=1  precision=Full  arith_type=Unsigned  n_bits=16  bin_pt=14  quantization=Truncate  overflow=Wrap  use_behavioral_HDL=off  hw_selection=Fabric  pipelined=off  XmcBlockStatus=1  maskContainerNames=tabcontainer1  block_type=addsub  block_config=sysgen:Addsub_config
  re0*re1 : hdlBasic/Mult  precision=Full  arith_type="Signed  (2's comp)"  n_bits=16  bin_pt=14  quantization=Truncate  overflow=Wrap  en=off  latency=3  use_behavioral_HDL=off  opt=Speed  use_embedded=on  optimum_pipeline=off  pipeline=on  use_rpm=on  placement_style=Triangular  XmcBlockStatus=1  maskContainerNames=group1  block_type=mult  block_config=sysgen:Mult_config  block_width=598  block_height=876
  re0*re1+im0*im1 : hdlBasic/AddSub  mode=Addition  use_carryin=off  use_carryout=off  en=off  latency=1  precision=Full  arith_type=Unsigned  n_bits=16  bin_pt=14  quantization=Truncate  overflow=Wrap  use_behavioral_HDL=off  hw_selection=Fabric  pipelined=off  XmcBlockStatus=1  maskContainerNames=tabcontainer1  block_type=addsub  block_config=sysgen:Addsub_config
  re1*im0 : hdlBasic/Mult  precision=Full  arith_type="Signed  (2's comp)"  n_bits=16  bin_pt=14  quantization=Truncate  overflow=Wrap  en=off  latency=3  use_behavioral_HDL=off  opt=Speed  use_embedded=on  optimum_pipeline=off  pipeline=on  use_rpm=on  placement_style=Triangular  XmcBlockStatus=1  maskContainerNames=group1  block_type=mult  block_config=sysgen:Mult_config  block_width=598  block_height=876
  Z : Outport
  wires:
  In3/1 -> re1*im0/2, im0*im1/1
  re0*im1-re1*im0/1 -> CORDIC ATAN/2(y)
  In2/1 -> re0*re1/2, re1*im0/1
  In4/1 -> re0*im1/2, im0*im1/2
  re0*im1/1 -> re0*im1-re1*im0/1
  In1/1 -> re0*im1/1, re0*re1/1
  re0*re1/1 -> re0*re1+im0*im1/1
  im0*im1/1 -> re0*re1+im0*im1/2
  re0*re1+im0*im1/1 -> CORDIC ATAN/1(x)
  re1*im0/1 -> re0*im1-re1*im0/2
  CORDIC ATAN/2(Z) -> Z/1

== system kay1024_recursive_demo/Subsystem/Subsystem16/Subsystem4 ==
  In1 : Inport
  In2 : Inport  Port=2
  In3 : Inport  Port=3
  In4 : Inport  Port=4
  CORDIC ATAN : Subsystem  mask(Xilinx CORDIC ATAN){stages=15, pe_nbits=30, pe_binpt=18, pipeline_x=ones(1,15), prev_stages=15, pipeline=[1  1  1  1  1  1  1  1  1  1  1  1  1  1  1]}
      mask prompts: stages "Number of Processing Elements (integer value starting from 1)"; pe_nbits "X, Y Data Width"; pe_binpt "X, Y Binary Point Position"; pipeline_x "Latency for each Processing Element [1 0 0 1]"; prev_stages "Previous Number of Stages"; pipeline "Previous Pipeline Values"
      mask help: A parallel implementation, circular vectoring mode CORDIC processor for performing rectangular-to-polar conversion. The number of iteration stages (and resultant output accuracy) and the processor arithmetic precision are controlled by the mask customization.
      mask init: same as kay1024_recursive_demo/Subsystem/Subsystem16/Subsystem/CORDIC ATAN
      settings: CopyFcn=set_param(gcb, 'MaskSelfModifiable', 'on', 'LinkStatus', 'none');
      mask Help: eval('');xlDoc('-book','sysgen','-topic','CORDIC_ATAN');
      mask Display:
      | patch([0 iWidth iWidth 0],[0 0 iHeight iHeight] , bg);
      | patch(logoX,logoY , fg);
      | text(iCx-6,iCy,'z');
      | text(iCx,iCy+4,str);
      | port_label('input',1,'x');
      | port_label('input',2,'y');
      | port_label('output',1,'mag');
      | port_label('output',2,'atan');
      | plot([0 0 iWidth iWidth 0], [0 iHeight iHeight 0 0]);
  im0*im1 : hdlBasic/Mult  precision=Full  arith_type="Signed  (2's comp)"  n_bits=16  bin_pt=14  quantization=Truncate  overflow=Wrap  en=off  latency=3  use_behavioral_HDL=off  opt=Speed  use_embedded=on  optimum_pipeline=off  pipeline=on  use_rpm=on  placement_style=Triangular  XmcBlockStatus=1  maskContainerNames=group1  block_type=mult  block_config=sysgen:Mult_config  block_width=598  block_height=876
  re0*im1 : hdlBasic/Mult  precision=Full  arith_type="Signed  (2's comp)"  n_bits=16  bin_pt=14  quantization=Truncate  overflow=Wrap  en=off  latency=3  use_behavioral_HDL=off  opt=Speed  use_embedded=on  optimum_pipeline=off  pipeline=on  use_rpm=on  placement_style=Triangular  XmcBlockStatus=1  maskContainerNames=group1  block_type=mult  block_config=sysgen:Mult_config  block_width=598  block_height=876
  re0*im1-re1*im0 : hdlBasic/AddSub  mode=Subtraction  use_carryin=off  use_carryout=off  en=off  latency=1  precision=Full  arith_type=Unsigned  n_bits=16  bin_pt=14  quantization=Truncate  overflow=Wrap  use_behavioral_HDL=off  hw_selection=Fabric  pipelined=off  XmcBlockStatus=1  maskContainerNames=tabcontainer1  block_type=addsub  block_config=sysgen:Addsub_config
  re0*re1 : hdlBasic/Mult  precision=Full  arith_type="Signed  (2's comp)"  n_bits=16  bin_pt=14  quantization=Truncate  overflow=Wrap  en=off  latency=3  use_behavioral_HDL=off  opt=Speed  use_embedded=on  optimum_pipeline=off  pipeline=on  use_rpm=on  placement_style=Triangular  XmcBlockStatus=1  maskContainerNames=group1  block_type=mult  block_config=sysgen:Mult_config  block_width=598  block_height=876
  re0*re1+im0*im1 : hdlBasic/AddSub  mode=Addition  use_carryin=off  use_carryout=off  en=off  latency=1  precision=Full  arith_type=Unsigned  n_bits=16  bin_pt=14  quantization=Truncate  overflow=Wrap  use_behavioral_HDL=off  hw_selection=Fabric  pipelined=off  XmcBlockStatus=1  maskContainerNames=tabcontainer1  block_type=addsub  block_config=sysgen:Addsub_config
  re1*im0 : hdlBasic/Mult  precision=Full  arith_type="Signed  (2's comp)"  n_bits=16  bin_pt=14  quantization=Truncate  overflow=Wrap  en=off  latency=3  use_behavioral_HDL=off  opt=Speed  use_embedded=on  optimum_pipeline=off  pipeline=on  use_rpm=on  placement_style=Triangular  XmcBlockStatus=1  maskContainerNames=group1  block_type=mult  block_config=sysgen:Mult_config  block_width=598  block_height=876
  Z : Outport
  wires:
  In3/1 -> re1*im0/2, im0*im1/1
  re0*im1-re1*im0/1 -> CORDIC ATAN/2(y)
  In2/1 -> re0*re1/2, re1*im0/1
  In4/1 -> re0*im1/2, im0*im1/2
  re0*im1/1 -> re0*im1-re1*im0/1
  In1/1 -> re0*im1/1, re0*re1/1
  re0*re1/1 -> re0*re1+im0*im1/1
  im0*im1/1 -> re0*re1+im0*im1/2
  re0*re1+im0*im1/1 -> CORDIC ATAN/1(x)
  re1*im0/1 -> re0*im1-re1*im0/2
  CORDIC ATAN/2(Z) -> Z/1

== system kay1024_recursive_demo/Subsystem/Subsystem16/Subsystem5 ==
  In1 : Inport
  In2 : Inport  Port=2
  In3 : Inport  Port=3
  In4 : Inport  Port=4
  CORDIC ATAN : Subsystem  mask(Xilinx CORDIC ATAN){stages=15, pe_nbits=30, pe_binpt=18, pipeline_x=ones(1,15), prev_stages=15, pipeline=[1  1  1  1  1  1  1  1  1  1  1  1  1  1  1]}
      mask prompts: stages "Number of Processing Elements (integer value starting from 1)"; pe_nbits "X, Y Data Width"; pe_binpt "X, Y Binary Point Position"; pipeline_x "Latency for each Processing Element [1 0 0 1]"; prev_stages "Previous Number of Stages"; pipeline "Previous Pipeline Values"
      mask help: A parallel implementation, circular vectoring mode CORDIC processor for performing rectangular-to-polar conversion. The number of iteration stages (and resultant output accuracy) and the processor arithmetic precision are controlled by the mask customization.
      mask init: same as kay1024_recursive_demo/Subsystem/Subsystem16/Subsystem/CORDIC ATAN
      settings: CopyFcn=set_param(gcb, 'MaskSelfModifiable', 'on', 'LinkStatus', 'none');
      mask Help: eval('');xlDoc('-book','sysgen','-topic','CORDIC_ATAN');
      mask Display:
      | patch([0 iWidth iWidth 0],[0 0 iHeight iHeight] , bg);
      | patch(logoX,logoY , fg);
      | text(iCx-6,iCy,'z');
      | text(iCx,iCy+4,str);
      | port_label('input',1,'x');
      | port_label('input',2,'y');
      | port_label('output',1,'mag');
      | port_label('output',2,'atan');
      | plot([0 0 iWidth iWidth 0], [0 iHeight iHeight 0 0]);
  im0*im1 : hdlBasic/Mult  precision=Full  arith_type="Signed  (2's comp)"  n_bits=16  bin_pt=14  quantization=Truncate  overflow=Wrap  en=off  latency=3  use_behavioral_HDL=off  opt=Speed  use_embedded=on  optimum_pipeline=off  pipeline=on  use_rpm=on  placement_style=Triangular  XmcBlockStatus=1  maskContainerNames=group1  block_type=mult  block_config=sysgen:Mult_config  block_width=598  block_height=876
  re0*im1 : hdlBasic/Mult  precision=Full  arith_type="Signed  (2's comp)"  n_bits=16  bin_pt=14  quantization=Truncate  overflow=Wrap  en=off  latency=3  use_behavioral_HDL=off  opt=Speed  use_embedded=on  optimum_pipeline=off  pipeline=on  use_rpm=on  placement_style=Triangular  XmcBlockStatus=1  maskContainerNames=group1  block_type=mult  block_config=sysgen:Mult_config  block_width=598  block_height=876
  re0*im1-re1*im0 : hdlBasic/AddSub  mode=Subtraction  use_carryin=off  use_carryout=off  en=off  latency=1  precision=Full  arith_type=Unsigned  n_bits=16  bin_pt=14  quantization=Truncate  overflow=Wrap  use_behavioral_HDL=off  hw_selection=Fabric  pipelined=off  XmcBlockStatus=1  maskContainerNames=tabcontainer1  block_type=addsub  block_config=sysgen:Addsub_config
  re0*re1 : hdlBasic/Mult  precision=Full  arith_type="Signed  (2's comp)"  n_bits=16  bin_pt=14  quantization=Truncate  overflow=Wrap  en=off  latency=3  use_behavioral_HDL=off  opt=Speed  use_embedded=on  optimum_pipeline=off  pipeline=on  use_rpm=on  placement_style=Triangular  XmcBlockStatus=1  maskContainerNames=group1  block_type=mult  block_config=sysgen:Mult_config  block_width=598  block_height=876
  re0*re1+im0*im1 : hdlBasic/AddSub  mode=Addition  use_carryin=off  use_carryout=off  en=off  latency=1  precision=Full  arith_type=Unsigned  n_bits=16  bin_pt=14  quantization=Truncate  overflow=Wrap  use_behavioral_HDL=off  hw_selection=Fabric  pipelined=off  XmcBlockStatus=1  maskContainerNames=tabcontainer1  block_type=addsub  block_config=sysgen:Addsub_config
  re1*im0 : hdlBasic/Mult  precision=Full  arith_type="Signed  (2's comp)"  n_bits=16  bin_pt=14  quantization=Truncate  overflow=Wrap  en=off  latency=3  use_behavioral_HDL=off  opt=Speed  use_embedded=on  optimum_pipeline=off  pipeline=on  use_rpm=on  placement_style=Triangular  XmcBlockStatus=1  maskContainerNames=group1  block_type=mult  block_config=sysgen:Mult_config  block_width=598  block_height=876
  Z : Outport
  wires:
  In3/1 -> re1*im0/2, im0*im1/1
  re0*im1-re1*im0/1 -> CORDIC ATAN/2(y)
  In2/1 -> re0*re1/2, re1*im0/1
  In4/1 -> re0*im1/2, im0*im1/2
  re0*im1/1 -> re0*im1-re1*im0/1
  In1/1 -> re0*im1/1, re0*re1/1
  re0*re1/1 -> re0*re1+im0*im1/1
  im0*im1/1 -> re0*re1+im0*im1/2
  re0*re1+im0*im1/1 -> CORDIC ATAN/1(x)
  re1*im0/1 -> re0*im1-re1*im0/2
  CORDIC ATAN/2(Z) -> Z/1
